simulink model "VirtualVehicle_Lab2_Soln"  (R2023b)
settings: Solver=VariableStepAuto  StartTime=0.0  StopTime=30  MaxStep=0.002  RelTol=1e-3
values from neighbouring files (symbols this model uses):
  m = 1000    [VehicleModelSoln.m]
  s = tf('s')    [PositionAnalysisSoln.m]
undefined symbols (not defined in the file or in its folder): X, Y, Z
libraries: sm_lib x59, nesl_utility x12, fl_lib x5, sdl_lib x1
(part 1 of 2)
settings Model: Creator=Rocksmithed  LastModifiedBy=callie
settings DebuggingCC: UnconnectedInputMsg=warning  UnconnectedOutputMsg=warning  UnconnectedLineMsg=warning
settings ModelReferenceCC: EnableRefExpFcnMdlSchedulingChecks=on
settings RTWCC: DLArmComputeVersion=19.05
settings SimscapeCC: SimscapeLogType=all  SimscapeLogLimitData=off
settings DiagnosticsConfigSet: SimMechanicsConflictingReferenceFrames=none
settings ExplorerConfigSet: InternalSimMechanicsExplorerSettings="<ExplorerConfiguration><canonicalview>default</canonicalview><AnimationSetting><BasePlaybackSpeed>1.0</BasePlaybackSpeed><PlaybackSpeedFactor>1.0</PlaybackSpeedFactor></AnimationSetting><TilePanel><TileInfo><Tiles Columns=\"1\" Count=\"2\" Rows=\"2\"><Column Weight=\"1\"/><Row Weight=\"0.4997\"/><Row Weight=\"0.5003\"/><Tile Height=\"1\" Width=\"1\" X=\"0\" Y=\"0\"/><Tile Height=\"1\" Width=\"1\" X=\"0\" Y=\"1\"/></Tiles></TileInfo><SceneInfo><SceneViewer><BGColor><R>0.800000011920928955</R><G>0.800000011920928955</G><B>0.800000011920928955</B></BGColor><Camera><DoPerspective>on</DoPerspective><Position><X>5.90000000000000036</X><Y>-6</Y><Z>6.75</Z></Position><Center><X>5.32642356364895431</X><Y>-5.37249312840286741</Y><Z>6.22345921548163616</Z></Center><Up><X>0</X><Y>0</Y><Z>1</Z></Up><ViewLimDist>1</ViewLimDist><YLim>0.466307658154998583</YLim><XLim>1.21820086771592928</XLim></Camera></SceneViewer><SceneViewer><BGColor><R>0.800000011920928955</R><G>0.800000011920928955</G><B>0.800000011920928955</B></BGColor><Camera><DoPerspective>on</DoPerspective><Position><X>-1</X><Y>-15</Y><Z>0</Z></Position><Center><X>-1</X><Y>-14</Y><Z>-2.22044604925031308e-16</Z></Center><Up><X>0</X><Y>0</Y><Z>1</Z></Up><ViewLimDist>1</ViewLimDist><YLim>0.466307658154998583</YLim><XLim>1.21239991120299639</XLim></Camera></SceneViewer></SceneInfo></TilePanel><MechEditorPanel><Cameras><Camera><Id>Camera1</Id><Value><Name>Camera Tracking Iso</Name><NativeCamera><PositionTrackingFeature>Vehicle_and_road.Animation.Cameras.Reference_Camera_Iso.R</PositionTrackingFeature><CenterTrackingFeature>Vehicle_and_road.Animation.Cameras.Reference_Camera_Iso.R</CenterTrackingFeature><UpVectorTrackingFeature>Vehicle_and_road.Animation.World_Frame.W</UpVectorTrackingFeature><CenterTrackingOrigin>off</CenterTrackingOrigin><CenterTrackingDirection>-Z</CenterTrackingDirection><UpVectorTrackingDirection>+Z</UpVectorTrackingDirection></NativeCamera></Value></Camera><Camera><Id>Camera2</Id><Value><Name>Camera Tracking Side</Name><NativeCamera><PositionTrackingFeature>Vehicle_and_road.Animation.Cameras.Reference_Camera_Side.R</PositionTrackingFeature><CenterTrackingFeature>Vehicle_and_road.Animation.Cameras.Reference_Camera_Side.R</CenterTrackingFeature><UpVectorTrackingFeature>Vehicle_and_road.Animation.World_Frame.W</UpVectorTrackingFeature><CenterTrackingOrigin>off</CenterTrackingOrigin><CenterTrackingDirection>-Z</CenterTrackingDirection><UpVectorTrackingDirection>+Z</UpVectorTrackingDirection></NativeCamera></Value></Camera></Cameras><GfxPanelCameraMap><MapElement CameraMLId=\"Camera1\" GfxPanelIndex=\"0\"/><MapElement CameraMLId=\"Camera2\" GfxPanelIndex=\"1\"/></GfxPanelCameraMap><VideoCreator><PlaybackSpeedRatio>1.0</PlaybackSpeedRatio><FrameRate>30</FrameRate><VideoFormat>Motion JPEG AVI</VideoFormat><FrameSize>auto</FrameSize></VideoCreator></MechEditorPanel></ExplorerConfiguration>"

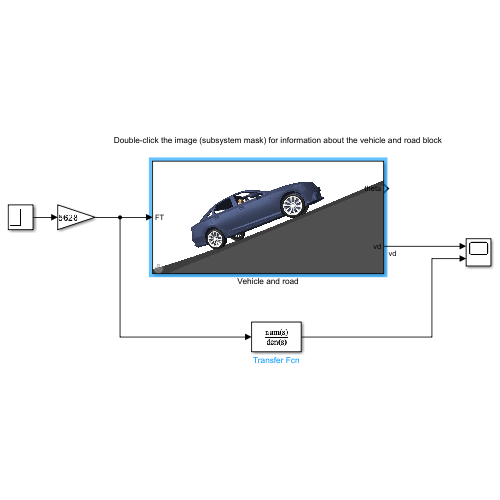
[thumbnail: Simulink's stored preview of the top-level diagram]
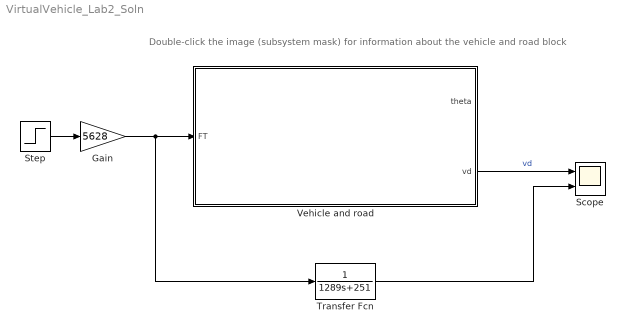
== system VirtualVehicle_Lab2_Soln ==
  note: Double-click the image (subsystem mask) for information about the vehicle and road block
  Gain : Gain  Gain=5628
  Scope : Scope  NumInputPorts=2
  Step : Step  Time=0  SampleTime=0
  Transfer Fcn : TransferFcn  Denominator=[1289 251]
  Vehicle and road : Subsystem  mask{MaxF=14800.0, brkok=on, dtype=none, randbumps=on, h=20.0, bumpspace=68.0}
      mask prompts: MaxF "Traction force saturation limit"; brkok "Allow braking"; dtype "Disturbance type"; randbumps "Randomize bumps"; h "Disturbance height (m)"; bumpspace "Bump spacing (m)"
      mask help:
      | This block provides a 2D implementation and visualization of a virtual vehicle.
      |
      | Inputs:
      |    FT: traction force in Newtons.
      | Outputs:
      |    theta: road grade at current position in radians.
      |    vd: velocity in the direction of travel in m/s (car frame).
      mask init:
      | L = 500; % Track length (meters)
      | tw = 10; % Transition width (meters)
      | ext = 600; % Extra at the end
      | depth = 0.25; % Road depth (meters)
      | N = 10e3;
      | 
      | roadw = 5; % road width (m)
      | 
      | markerFreq = 200; % marker every X points
      | markerw = 0.1; % marker width
      | markerd = 0.05; % marker depth
      | markerh = 1.5; % marker height
      | 
      | b_friction = 250; % Additional friction force coefficient (N*s/m)
      | 
      | if(dtype==2)
      |     xb = [-4,L/4,L/2-tw,...
      |       L/2+tw,L*3/4,L+ext];
      |     yf = @(x) (x > L/4).*(x < L/2).*((h/(L/4)).*(x-L/4)) ...
      |         + (x >= L/2).*(x < 3*L/4).*((-h/(L/4)).*(x-L/2) + h);
      |     yb = yf(xb);
      | 
      | elseif(dtype==3)
      |     bumpx = L/10:bumpspace/2:9*L/10;
      |     n = 1:numel(bumpx);
      |     xb = [-4,bumpx,L,L+ext];
      |     yb = [0,h/2*(1+(-1).^(n)),0,0];
      | 
      |     % Bump randomization
      |     if(randbumps)
      |         bh = rand(1,numel(bumpx)).*h/2.*(1+(-1).^(n));
      |         yb = [0,bh,0,0];
      |     end
      | 
      | else
      |     xb = [-4,L+ext];
      |     yb = xb*0;
      |     
      | end
      |     
      | % Vehicle position
      | xc = linspace(0,xb(end),N);
      | yc = pchip([0,xb(2:end)],[0,yb(2:end)],xc);
      | 
      | % Road position
      | x = linspace(xb(1),xb(end),N);
      | y = pchip(xb,yb,x);
      | x2 = [x(1),x,x(end)];
      | y2 = [-depth,y,-depth];
      | roadcs = [x2(end:-1:1);y2(end:-1:1)]';
      | 
      | % Markers
      | ix = 1:round(markerFreq):length(x);
      | xm1 = [x(ix)-markerd;x(ix)-markerd;x(ix)+markerd;x(ix)+markerd];
      | ym1 = [y(ix)*0;y(ix)+markerh;y(ix)+markerh;y(ix)*0];
      | xm = [xm1(1),xm1(:)',xm1(end)];
      | ym = [-depth,ym1(:)',-depth];
      | 
      | markercs = [xm(end:-1:1);ym(end:-1:1)]';
      | 
      | 
      | % Braking?
      | llim = 0;
      | if(brkok)
      |     llim = -inf;
      | end
      mask TypeOptions dtype: none | hill | bumps
      mask DialogControl Container3 Prompt: Vehicle
      mask DialogControl Container4 Prompt: Road
      mask Display: image('vehicle.png');
  wires:
  Step/1 -> Gain/1
  Vehicle and road/2(vd) -> Scope/1  "vd"
  Transfer Fcn/1 -> Scope/2
  Gain/1 -> Transfer Fcn/1, Vehicle and road/1(FT)

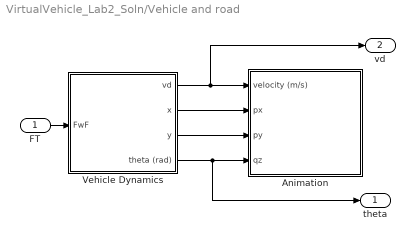
== system VirtualVehicle_Lab2_Soln/Vehicle and road ==
  FT : Inport
  Animation : Subsystem
  Vehicle Dynamics : Subsystem
  theta : Outport
  vd : Outport  Port=2
  wires:
  Vehicle Dynamics/1(vd) -> vd/1, Animation/1(velocity (m/s))
  FT/1 -> Vehicle Dynamics/1(FwF)
  Vehicle Dynamics/4(theta (rad)) -> theta/1, Animation/4(qz)
  Vehicle Dynamics/2(x) -> Animation/2(px)
  Vehicle Dynamics/3(y) -> Animation/3(py)

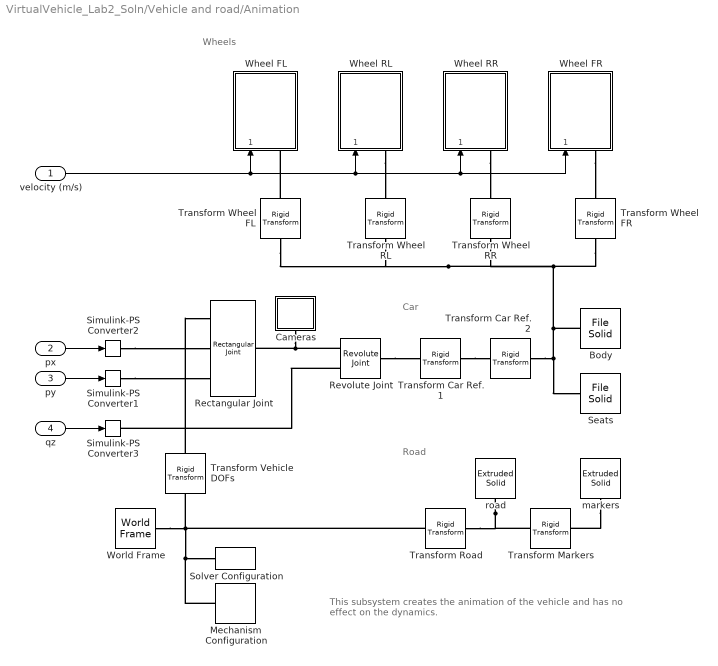
== system VirtualVehicle_Lab2_Soln/Vehicle and road/Animation ==
  note: This subsystem creates the animation of the vehicle and has no effect on the dynamics.
  note: Car
  note: Wheels
  note: Road
  velocity (m/s) : Inport
  px : Inport  Port=2
  py : Inport  Port=3
  qz : Inport  Port=4
  Body : sm_lib/Body Elements/File Solid  ExtGeomFileName=cc_Sedan_Hamba_body.STL  UnitType=Custom  ExtGeomFileUnits=mm  StepReaderType=HEX  ExportConvexHullGeometry=off  InertiaType=CalculateFromGeometry  Mass=1  MassUnits=kg  CenterOfMass=[0 0 0]  CenterOfMassUnits=m  MomentsOfInertia=[1 1 1]  MomentsOfInertiaUnits=kg*m^2  ProductsOfInertia=[0 0 0]  ProductsOfInertiaUnits=kg*m^2  BasedOnType=Density  Density=1000  DensityUnits=kg/m^3  DoExposeReferenceFrame=on  SerializedFrames=<Frames/>  GraphicType=FromGeometry  MarkerShape=Sphere  MarkerSize=10  GraphicVisPropType=AdvancedVisualProperties  GraphicDiffuseColor="[0.2670    0.3060    0.4270]"  GraphicSpecularColor="[0.2670    0.3060    0.4270]"  GraphicAmbientColor="[0.2670    0.3060    0.4270]/3"  GraphicEmissiveColor=[0 0 0]  GraphicShininess=20  GraphicOpacity=1.0
  Cameras : Subsystem
  Mechanism Configuration : sm_lib/Utilities/Mechanism Configuration  UniformGravity=Constant  GravityVector=[0 0 -9.80665*0]  GravityVectorUnits=m/s^2  GravityUnits=m/s^2  LinearizationDelta=0.001  JointModeTransitionNonlinearIterations=2
  Rectangular Joint : sm_lib/Joints/Rectangular Joint  JointMode=Normal  SenseConstraintForce=off  SenseConstraintForceX=off  SenseConstraintForceY=off  SenseConstraintForceZ=off  SenseConstraintTorque=off  SenseConstraintTorqueX=off  SenseConstraintTorqueY=off  SenseConstraintTorqueZ=off  SenseTotalForce=off  SenseTotalForceX=off  SenseTotalForceY=off  SenseTotalForceZ=off  SenseTotalTorque=off  SenseTotalTorqueX=off  SenseTotalTorqueY=off  SenseTotalTorqueZ=off  CompositeWrenchDir=FollowerOnBase  CompositeWrenchFrame=BaseFrame  PxEquilibriumPosition=0  PxEquilibriumPositionUnits=m  PxSpringStiffness=0  PxSpringStiffnessUnits=N/m  PxDampingCoefficient=0  PxDampingCoefficientUnits=N/(m/s)  PxTorqueActuationMode=ComputedTorque  PxMotionActuationMode=InputMotion  PxSensePosition=off  PxSenseVelocity=off  PxSenseAcceleration=off  PxSenseTorqueForce=off  PxSenseLowerLimitTorqueForce=off  PxSenseUpperLimitTorqueForce=off  PxLowerLimitSpecify=off  PxLowerLimitBound=-1  PxLowerLimitBoundUnits=m  PxLowerLimitStiffness=1e6  PxLowerLimitStiffnessUnits=N/m  PxLowerLimitDamping=1e3  PxLowerLimitDampingUnits=N/(m/s)  PxLowerLimitTransitionRegionWidth=1e-4  PxLowerLimitTransitionRegionWidthUnits=m  PxUpperLimitSpecify=off  PxUpperLimitBound=1  PxUpperLimitBoundUnits=m  PxUpperLimitStiffness=1e6  PxUpperLimitStiffnessUnits=N/m  PxUpperLimitDamping=1e3  PxUpperLimitDampingUnits=N/(m/s)  PxUpperLimitTransitionRegionWidth=1e-4  PxUpperLimitTransitionRegionWidthUnits=m  PxPositionTargetSpecify=off  PxPositionTargetPriority=High  PxPositionTargetValue=0  PxPositionTargetValueUnits=m  PxVelocityTargetSpecify=off  PxVelocityTargetPriority=High  PxVelocityTargetValue=0  PxVelocityTargetValueUnits=m/s  PyEquilibriumPosition=0  PyEquilibriumPositionUnits=m  PySpringStiffness=0  PySpringStiffnessUnits=N/m  PyDampingCoefficient=0  PyDampingCoefficientUnits=N/(m/s)  PyTorqueActuationMode=ComputedTorque  PyMotionActuationMode=InputMotion  PySensePosition=off  PySenseVelocity=off  PySenseAcceleration=off  PySenseTorqueForce=off  PySenseLowerLimitTorqueForce=off  PySenseUpperLimitTorqueForce=off  PyLowerLimitSpecify=off  PyLowerLimitBound=-1  PyLowerLimitBoundUnits=m  PyLowerLimitStiffness=1e6  PyLowerLimitStiffnessUnits=N/m  PyLowerLimitDamping=1e3  PyLowerLimitDampingUnits=N/(m/s)  PyLowerLimitTransitionRegionWidth=1e-4  PyLowerLimitTransitionRegionWidthUnits=m  PyUpperLimitSpecify=off  PyUpperLimitBound=1  PyUpperLimitBoundUnits=m  PyUpperLimitStiffness=1e6  PyUpperLimitStiffnessUnits=N/m  PyUpperLimitDamping=1e3  PyUpperLimitDampingUnits=N/(m/s)  PyUpperLimitTransitionRegionWidth=1e-4  PyUpperLimitTransitionRegionWidthUnits=m  PyPositionTargetSpecify=off  PyPositionTargetPriority=High  PyPositionTargetValue=0  PyPositionTargetValueUnits=m  PyVelocityTargetSpecify=off  PyVelocityTargetPriority=High  PyVelocityTargetValue=0  PyVelocityTargetValueUnits=m/s
  Revolute Joint : sm_lib/Joints/Revolute Joint  JointMode=Normal  SenseConstraintForce=off  SenseConstraintForceX=off  SenseConstraintForceY=off  SenseConstraintForceZ=off  SenseConstraintTorque=off  SenseConstraintTorqueX=off  SenseConstraintTorqueY=off  SenseConstraintTorqueZ=off  SenseTotalForce=off  SenseTotalForceX=off  SenseTotalForceY=off  SenseTotalForceZ=off  SenseTotalTorque=off  SenseTotalTorqueX=off  SenseTotalTorqueY=off  SenseTotalTorqueZ=off  CompositeWrenchDir=FollowerOnBase  CompositeWrenchFrame=BaseFrame  EquilibriumPosition=0  EquilibriumPositionUnits=deg  SpringStiffness=0  SpringStiffnessUnits=N*m/deg  DampingCoefficient=0  DampingCoefficientUnits=N*m/(deg/s)  TorqueActuationMode=ComputedTorque  MotionActuationMode=InputMotion  SensePosition=off  SenseVelocity=off  SenseAcceleration=off  SenseTorqueForce=off  SenseLowerLimitTorqueForce=off  SenseUpperLimitTorqueForce=off  LowerLimitSpecify=off  LowerLimitBound=-90  LowerLimitBoundUnits=deg  LowerLimitStiffness=1e4  LowerLimitStiffnessUnits=N*m/deg  LowerLimitDamping=10  LowerLimitDampingUnits=N*m/(deg/s)  LowerLimitTransitionRegionWidth=0.1  LowerLimitTransitionRegionWidthUnits=deg  UpperLimitSpecify=off  UpperLimitBound=90  UpperLimitBoundUnits=deg  UpperLimitStiffness=1e4  UpperLimitStiffnessUnits=N*m/deg  UpperLimitDamping=10  UpperLimitDampingUnits=N*m/(deg/s)  UpperLimitTransitionRegionWidth=0.1  UpperLimitTransitionRegionWidthUnits=deg  PositionTargetSpecify=off  PositionTargetPriority=High  PositionTargetValue=0  PositionTargetValueUnits=deg  VelocityTargetSpecify=off  VelocityTargetPriority=High  VelocityTargetValue=0  VelocityTargetValueUnits=deg/s
  Seats : sm_lib/Body Elements/File Solid  ExtGeomFileName=cc_Sedan_Hamba_seats.STL  UnitType=Custom  ExtGeomFileUnits=mm  StepReaderType=HEX  ExportConvexHullGeometry=off  InertiaType=CalculateFromGeometry  Mass=1  MassUnits=kg  CenterOfMass=[0 0 0]  CenterOfMassUnits=m  MomentsOfInertia=[1 1 1]  MomentsOfInertiaUnits=kg*m^2  ProductsOfInertia=[0 0 0]  ProductsOfInertiaUnits=kg*m^2  BasedOnType=Density  Density=1000  DensityUnits=kg/m^3  DoExposeReferenceFrame=on  SerializedFrames=<Frames/>  GraphicType=FromGeometry  MarkerShape=Sphere  MarkerSize=10  GraphicVisPropType=SimpleVisualProperties  GraphicDiffuseColor="[0.98 0.74  0.52]"  GraphicSpecularColor="[1    0.9   0.8 1]"  GraphicAmbientColor=[0.15 0.05 0.05 1]  GraphicEmissiveColor=[0.0 0.0 0.0 1.0]  GraphicShininess=25  GraphicOpacity=1.0
  Simulink-PS Converter1 : nesl_utility/Simulink-PS Converter  PhysicalDomain=network_engine_domain  SubClassName=ps_input  LeftPortType=input  RightPortType=output  PseudoPeriodic=off  Frequencies=[]  NoiseDistribution=none  NoiseParameters=[]  Unit=1  AffineConversion=off  FilteringAndDerivatives=filter  SimscapeFilterOrder=2  InputFilterTimeConstant=0.001  UdotUserProvided=0
  Simulink-PS Converter2 : nesl_utility/Simulink-PS Converter  PhysicalDomain=network_engine_domain  SubClassName=ps_input  LeftPortType=input  RightPortType=output  PseudoPeriodic=off  Frequencies=[]  NoiseDistribution=none  NoiseParameters=[]  Unit=1  AffineConversion=off  FilteringAndDerivatives=filter  SimscapeFilterOrder=2  InputFilterTimeConstant=0.001  UdotUserProvided=0
  Simulink-PS Converter3 : nesl_utility/Simulink-PS Converter  PhysicalDomain=network_engine_domain  SubClassName=ps_input  LeftPortType=input  RightPortType=output  PseudoPeriodic=off  Frequencies=[]  NoiseDistribution=none  NoiseParameters=[]  Unit=rad  AffineConversion=off  FilteringAndDerivatives=filter  SimscapeFilterOrder=2  InputFilterTimeConstant=0.001  UdotUserProvided=0
  Solver Configuration : nesl_utility/Solver Configuration  PhysicalDomain=network_engine_domain  SubClassName=solver  LeftPortType=input  RightPortType=generic  Tones=[]  Harmonics=[]  SimulateNoise=off  Profile=off  UseLocalSampling=off  EnableSwitchedLinearOptims=on  FrequencyDomain=off  UseCCode=off  RelTol=0.001  AbsTol=1e-06  MinStep=1e-09  ToWorkspace=off  RevertToSquareIcSolve=off  NumHomotopyIterations=100  PhasorMode=off  PhasorModeNumHarmonics=1  DoDC=off  ResidualTolerance=1e-09  UseLocalSolver=off  LocalSolverChoice=NE_BACKWARD_EULER_ADVANCER  LocalSolverSampleTime=0.001  DoFixedCost=off  MaxNonlinIter=3  MaxModeIter=2  ComputeImpulses=off  ImpulseIterations=2  LinearAlgebra=Sparse  EquationFormulation=NE_TIME_EF  DelaysMemoryBudget=1024  AutomaticFiltering=on  FilteringTimeConstant=0.001  PartitionStorageMethod=AS_NEEDED  PartitionMemoryBudget=1024  PartitionMethod=FAST
  Transform Car Ref. 1 : sm_lib/Frames and Transforms/Rigid Transform  TranslationMethod=None  TranslationStandardOffset=0  TranslationLengthUnit=m  TranslationStandardAxis=+Z  TranslationCartesianOffset=[0 0 0]  TranslationROffset=0  TranslationROffsetUnits=m  TranslationZOffset=0  TranslationZOffsetUnits=m  TranslationThetaOffset=0  TranslationThetaOffsetUnits=deg  RotationMethod=AlignedAxes  RotationAngleUnits=deg  RotationStandardAxis=+Z  RotationAngle=0.0  RotationArbitraryAxis=[0 0 1]  FollAlignAxisA=+Y  BaseAlignAxisA=+Z  FollAlignAxisB=+X  BaseAlignAxisB=+X  RotationSequenceAxes=FollowerAxes  RotationSequence=XYX  RotationSequenceAngles=[0 0 0]  RotationSequenceAnglesUnits=deg  RotationMatrix=[1 0 0; 0 1 0; 0 0 1]
  Transform Car Ref. 2 : sm_lib/Frames and Transforms/Rigid Transform  TranslationMethod=Cartesian  TranslationStandardOffset=0  TranslationLengthUnit=m  TranslationStandardAxis=+Z  TranslationCartesianOffset=[-4.1 -2 -3.25]  TranslationROffset=0  TranslationROffsetUnits=m  TranslationZOffset=0  TranslationZOffsetUnits=m  TranslationThetaOffset=0  TranslationThetaOffsetUnits=deg  RotationMethod=None  RotationAngleUnits=deg  RotationStandardAxis=+Z  RotationAngle=0.0  RotationArbitraryAxis=[0 0 1]  FollAlignAxisA=+X  BaseAlignAxisA=+Y  FollAlignAxisB=+Y  BaseAlignAxisB=+Z  RotationSequenceAxes=FollowerAxes  RotationSequence=XYX  RotationSequenceAngles=[0 0 0]  RotationSequenceAnglesUnits=deg  RotationMatrix=[1 0 0; 0 1 0; 0 0 1]
  Transform Markers : sm_lib/Frames and Transforms/Rigid Transform  TranslationMethod=StandardAxis  TranslationStandardOffset=-roadw/2-markerw  TranslationLengthUnit=m  TranslationStandardAxis=+Z  TranslationCartesianOffset=[0 0 0]  TranslationROffset=0  TranslationROffsetUnits=m  TranslationZOffset=0  TranslationZOffsetUnits=m  TranslationThetaOffset=0  TranslationThetaOffsetUnits=deg  RotationMethod=None  RotationAngleUnits=deg  RotationStandardAxis=+Z  RotationAngle=0.0  RotationArbitraryAxis=[0 0 1]  FollAlignAxisA=+X  BaseAlignAxisA=+Y  FollAlignAxisB=+Y  BaseAlignAxisB=+Z  RotationSequenceAxes=FollowerAxes  RotationSequence=XYX  RotationSequenceAngles=[0 0 0]  RotationSequenceAnglesUnits=deg  RotationMatrix=[1 0 0; 0 1 0; 0 0 1]
  Transform Road : sm_lib/Frames and Transforms/Rigid Transform  TranslationMethod=Cartesian  TranslationStandardOffset=0  TranslationLengthUnit=m  TranslationStandardAxis=+Z  TranslationCartesianOffset=[0 0 0]  TranslationROffset=0  TranslationROffsetUnits=m  TranslationZOffset=0  TranslationZOffsetUnits=m  TranslationThetaOffset=0  TranslationThetaOffsetUnits=deg  RotationMethod=AlignedAxes  RotationAngleUnits=deg  RotationStandardAxis=+Z  RotationAngle=0.0  RotationArbitraryAxis=[0 0 1]  FollAlignAxisA=+Z  BaseAlignAxisA=-Y  FollAlignAxisB=+Y  BaseAlignAxisB=+Z  RotationSequenceAxes=FollowerAxes  RotationSequence=XYX  RotationSequenceAngles=[0 0 0]  RotationSequenceAnglesUnits=deg  RotationMatrix=[1 0 0; 0 1 0; 0 0 1]
  Transform Vehicle DOFs : sm_lib/Frames and Transforms/Rigid Transform  TranslationMethod=Cartesian  TranslationStandardOffset=0  TranslationLengthUnit=m  TranslationStandardAxis=+Z  TranslationCartesianOffset=[0 0 0]  TranslationROffset=0  TranslationROffsetUnits=m  TranslationZOffset=0  TranslationZOffsetUnits=m  TranslationThetaOffset=0  TranslationThetaOffsetUnits=deg  RotationMethod=AlignedAxes  RotationAngleUnits=deg  RotationStandardAxis=+Z  RotationAngle=0.0  RotationArbitraryAxis=[0 0 1]  FollAlignAxisA=+Y  BaseAlignAxisA=+Z  FollAlignAxisB=+X  BaseAlignAxisB=+X  RotationSequenceAxes=FollowerAxes  RotationSequence=XYX  RotationSequenceAngles=[0 0 0]  RotationSequenceAnglesUnits=deg  RotationMatrix=[1 0 0; 0 1 0; 0 0 1]
  Transform Wheel FL : sm_lib/Frames and Transforms/Rigid Transform  TranslationMethod=None  TranslationStandardOffset=0  TranslationLengthUnit=m  TranslationStandardAxis=+Z  TranslationCartesianOffset=[0 0 0]  TranslationROffset=0  TranslationROffsetUnits=m  TranslationZOffset=0  TranslationZOffsetUnits=m  TranslationThetaOffset=0  TranslationThetaOffsetUnits=deg  RotationMethod=None  RotationAngleUnits=deg  RotationStandardAxis=+Z  RotationAngle=0.0  RotationArbitraryAxis=[0 0 1]  FollAlignAxisA=+X  BaseAlignAxisA=+Y  FollAlignAxisB=+Y  BaseAlignAxisB=+Z  RotationSequenceAxes=FollowerAxes  RotationSequence=XYX  RotationSequenceAngles=[0 0 0]  RotationSequenceAnglesUnits=deg  RotationMatrix=[1 0 0; 0 1 0; 0 0 1]
  Transform Wheel FR : sm_lib/Frames and Transforms/Rigid Transform  TranslationMethod=Cartesian  TranslationStandardOffset=0  TranslationLengthUnit=m  TranslationStandardAxis=+X  TranslationCartesianOffset=[8.22 4.4 0]  TranslationROffset=0  TranslationROffsetUnits=m  TranslationZOffset=0  TranslationZOffsetUnits=m  TranslationThetaOffset=0  TranslationThetaOffsetUnits=deg  RotationMethod=AlignedAxes  RotationAngleUnits=deg  RotationStandardAxis=+Z  RotationAngle=0.0  RotationArbitraryAxis=[0 0 1]  FollAlignAxisA=+Y  BaseAlignAxisA=-Y  FollAlignAxisB=+Z  BaseAlignAxisB=+Z  RotationSequenceAxes=FollowerAxes  RotationSequence=XYX  RotationSequenceAngles=[0 0 0]  RotationSequenceAnglesUnits=deg  RotationMatrix=[1 0 0; 0 1 0; 0 0 1]
  Transform Wheel RL : sm_lib/Frames and Transforms/Rigid Transform  TranslationMethod=Cartesian  TranslationStandardOffset=0  TranslationLengthUnit=m  TranslationStandardAxis=+Z  TranslationCartesianOffset=[-2.82 0 0]  TranslationROffset=0  TranslationROffsetUnits=m  TranslationZOffset=0  TranslationZOffsetUnits=m  TranslationThetaOffset=0  TranslationThetaOffsetUnits=deg  RotationMethod=None  RotationAngleUnits=deg  RotationStandardAxis=+Z  RotationAngle=0.0  RotationArbitraryAxis=[0 0 1]  FollAlignAxisA=+X  BaseAlignAxisA=+Y  FollAlignAxisB=+Y  BaseAlignAxisB=+Z  RotationSequenceAxes=FollowerAxes  RotationSequence=XYX  RotationSequenceAngles=[0 0 0]  RotationSequenceAnglesUnits=deg  RotationMatrix=[1 0 0; 0 1 0; 0 0 1]
  Transform Wheel RR : sm_lib/Frames and Transforms/Rigid Transform  TranslationMethod=Cartesian  TranslationStandardOffset=0  TranslationLengthUnit=m  TranslationStandardAxis=+X  TranslationCartesianOffset=[5.4 4.4 0]  TranslationROffset=0  TranslationROffsetUnits=m  TranslationZOffset=0  TranslationZOffsetUnits=m  TranslationThetaOffset=0  TranslationThetaOffsetUnits=deg  RotationMethod=AlignedAxes  RotationAngleUnits=deg  RotationStandardAxis=+Z  RotationAngle=0.0  RotationArbitraryAxis=[0 0 1]  FollAlignAxisA=+Y  BaseAlignAxisA=-Y  FollAlignAxisB=+Z  BaseAlignAxisB=+Z  RotationSequenceAxes=FollowerAxes  RotationSequence=XYX  RotationSequenceAngles=[0 0 0]  RotationSequenceAnglesUnits=deg  RotationMatrix=[1 0 0; 0 1 0; 0 0 1]
  Wheel FL : Subsystem
  Wheel FR : Subsystem
  Wheel RL : Subsystem
  Wheel RR : Subsystem
  World Frame : sm_lib/Frames and Transforms/World Frame
  markers : sm_lib/Body Elements/Extruded Solid  GraphicAmbientColor=[0.15 0.15 0.15 1.0]  BasedOnType=Density  CenterOfMass=[0 0 0]  CenterOfMassUnits=m  GraphicDiffuseColor=[1 0.9 0]  ExportConvexHullGeometry=off  ExtrusionCrossSection=markercs  ExtrusionCrossSectionUnits=m  Density=1000  DensityUnits=kg/m^3  DoExposeReferenceFrame=on  GraphicEmissiveColor=[0.0 0.0 0.0 1.0]  ExportEntireGeometry=off  ExtrusionLength=markerw  ExtrusionLengthUnits=m  ExtrusionType=General  SerializedFrames=<Frames/>  MarkerShape=Sphere  MarkerSize=10  GraphicType=FromGeometry  InertiaType=CalculateFromGeometry  Mass=1  MassUnits=kg  MomentsOfInertia=[1 1 1]  MomentsOfInertiaUnits=kg*m^2  PolygonNumSides=3  GraphicOpacity=1  PolygonOuterRadius=1  PolygonOuterRadiusUnits=m  ProductsOfInertia=[0 0 0]  ProductsOfInertiaUnits=kg*m^2  GraphicShininess=5  GraphicSpecularColor=[1 0.9 0]  GraphicVisPropType=SimpleVisualProperties
  road : sm_lib/Body Elements/Extruded Solid  GraphicAmbientColor=[0.15 0.15 0.15 1.0]  BasedOnType=Density  CenterOfMass=[0 0 0]  CenterOfMassUnits=m  GraphicDiffuseColor=[0.1 0.1 0.1]  ExportConvexHullGeometry=off  ExtrusionCrossSection=roadcs  ExtrusionCrossSectionUnits=m  Density=1000  DensityUnits=kg/m^3  DoExposeReferenceFrame=on  GraphicEmissiveColor=[0.0 0.0 0.0 1.0]  ExportEntireGeometry=off  ExtrusionLength=roadw  ExtrusionLengthUnits=m  ExtrusionType=General  SerializedFrames=<Frames/>  MarkerShape=Sphere  MarkerSize=10  GraphicType=FromGeometry  InertiaType=CalculateFromGeometry  Mass=1  MassUnits=kg  MomentsOfInertia=[1 1 1]  MomentsOfInertiaUnits=kg*m^2  PolygonNumSides=3  GraphicOpacity=1.0  PolygonOuterRadius=1  PolygonOuterRadiusUnits=m  ProductsOfInertia=[0 0 0]  ProductsOfInertiaUnits=kg*m^2  GraphicShininess=5  GraphicSpecularColor=[0.5 0.5 0.5 1.0]  GraphicVisPropType=AdvancedVisualProperties
  wires:
  velocity (m/s)/1 -> Wheel RL/1(velocity (m/s)), Wheel FR/1(velocity (m/s)), Wheel RR/1(velocity (m/s)), Wheel FL/1(velocity (m/s))
  px/1 -> Simulink-PS Converter2/1
  py/1 -> Simulink-PS Converter1/1
  qz/1 -> Simulink-PS Converter3/1
  connections:
  Wheel RL/LConn1 -- Transform Wheel RL/RConn1
  markers/RConn1 -- Transform Markers/RConn1
  Revolute Joint/LConn2 -- Simulink-PS Converter3/RConn1
  Wheel FR/LConn1 -- Transform Wheel FR/RConn1
  Wheel RR/LConn1 -- Transform Wheel RR/RConn1
  Revolute Joint/LConn1 -- Rectangular Joint/RConn1 -- Cameras/LConn1
  Transform Wheel FL/RConn1 -- Wheel FL/LConn1
  Transform Car Ref. 2/RConn1 -- Body/RConn1 -- Transform Wheel FR/LConn1 -- Transform Wheel FL/LConn1 -- Transform Wheel RL/LConn1 -- Transform Wheel RR/LConn1 -- Seats/RConn1
  World Frame/RConn1 -- Transform Road/LConn1 -- Mechanism Configuration/RConn1 -- Solver Configuration/RConn1 -- Transform Vehicle DOFs/LConn1
  road/RConn1 -- Transform Road/RConn1 -- Transform Markers/LConn1
  Transform Vehicle DOFs/RConn1 -- Rectangular Joint/LConn1
  Simulink-PS Converter2/RConn1 -- Rectangular Joint/LConn2
  Simulink-PS Converter1/RConn1 -- Rectangular Joint/LConn3
  Revolute Joint/RConn1 -- Transform Car Ref. 1/RConn1
  Transform Car Ref. 1/LConn1 -- Transform Car Ref. 2/LConn1

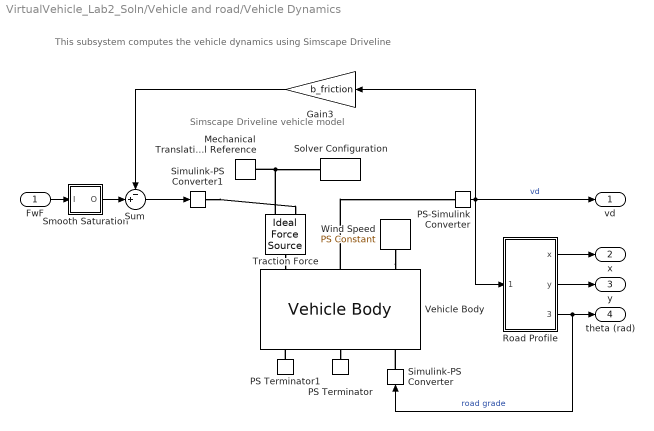
== system VirtualVehicle_Lab2_Soln/Vehicle and road/Vehicle Dynamics ==
  note: Simscape Driveline vehicle model
  note: This subsystem computes the vehicle dynamics using Simscape Driveline
  FwF : Inport
  Gain3 : Gain  Gain=b_friction
  Mechanical Translational Reference : fl_lib/Mechanical/Translational Elements/Mechanical Translational Reference
  PS Terminator : fl_lib/Physical Signals/Sinks/PS Terminator
  PS Terminator1 : fl_lib/Physical Signals/Sinks/PS Terminator
  PS-Simulink Converter : nesl_utility/PS-Simulink Converter  PhysicalDomain=network_engine_domain  SubClassName=ps_output  LeftPortType=input  RightPortType=output  PseudoPeriodic=off  Frequencies=[]  Unit=inherit  AffineConversion=off
  Road Profile : Subsystem
  Simulink-PS Converter : nesl_utility/Simulink-PS Converter  PhysicalDomain=network_engine_domain  SubClassName=ps_input  LeftPortType=input  RightPortType=output  PseudoPeriodic=off  Frequencies=[]  NoiseDistribution=none  NoiseParameters=[]  Unit=rad  AffineConversion=off  FilteringAndDerivatives=provide  SimscapeFilterOrder=1  InputFilterTimeConstant=0.001  UdotUserProvided=0
  Simulink-PS Converter1 : nesl_utility/Simulink-PS Converter  PhysicalDomain=network_engine_domain  SubClassName=ps_input  LeftPortType=input  RightPortType=output  PseudoPeriodic=off  Frequencies=[]  NoiseDistribution=none  NoiseParameters=[]  Unit=N  AffineConversion=off  FilteringAndDerivatives=provide  SimscapeFilterOrder=1  InputFilterTimeConstant=0.001  UdotUserProvided=0
  Smooth Saturation : Subsystem
  Solver Configuration : nesl_utility/Solver Configuration  PhysicalDomain=network_engine_domain  SubClassName=solver  LeftPortType=input  RightPortType=generic  Tones=[]  Harmonics=[]  SimulateNoise=off  Profile=off  UseLocalSampling=off  EnableSwitchedLinearOptims=on  FrequencyDomain=off  UseCCode=off  RelTol=0.001  AbsTol=1e-06  MinStep=1e-09  ToWorkspace=off  RevertToSquareIcSolve=off  NumHomotopyIterations=100  PhasorMode=off  PhasorModeNumHarmonics=1  DoDC=off  ResidualTolerance=1e-09  UseLocalSolver=off  LocalSolverChoice=NE_BACKWARD_EULER_ADVANCER  LocalSolverSampleTime=0.001  DoFixedCost=off  MaxNonlinIter=3  MaxModeIter=2  ComputeImpulses=off  ImpulseIterations=2  LinearAlgebra=auto  EquationFormulation=NE_TIME_EF  DelaysMemoryBudget=1024  AutomaticFiltering=on  FilteringTimeConstant=0.001  PartitionStorageMethod=AS_NEEDED  PartitionMemoryBudget=1024  PartitionMethod=ROBUST
  Sum : Sum  Inputs=-+|
  "Traction Force " : fl_lib/Mechanical/Mechanical Sources/Ideal Force Source
  Vehicle Body : sdl_lib/Tires & Vehicles/Vehicle Body  mass=1300 kg  n_w=2  x_f=1.4 m  x_r=1.8 m  y_c=.35 m  mass_var=simscape.enum.onoff.off  model_pitch=simscape.enum.onoff.off  inertia=4000 kg*m^2  suspension_model=sdl.enum.linearTLU.linear  k_f=1e4 N/m  b_f=1e4 N/(m/s)  k_r=1e4 N/m  b_r=1e4 N/(m/s)  k_f_TLU=[-2000, -1000, 0, 1000, 2000] N  x_f_TLU=[-.4, -.2, 0, .2, .4] m  b_f_TLU=[-200, -100, 0, 100, 200] N  v_f_TLU=[-4, -2, 0, 2, 4] m/s  k_r_TLU=[-2000, -1000, 0, 1000, 2000] N  x_r_TLU=[-.4, -.2, 0, .2, .4] m  b_r_TLU=[-200, -100, 0, 100, 200] N  v_r_TLU=[-4, -2, 0, 2, 4] m/s  interp_method=simscape.enum.interpolation.linear  extrap_method=simscape.enum.extrapolation.linear  model_hardstop=simscape.enum.onoff.off  upper_bound_f=.25 m  lower_bound_f=-.25 m  stop_k_f=1e6 N/m  stop_b_f=150 N/(m/s)  upper_bound_r=.25 m  lower_bound_r=-.25 m  stop_k_r=1e6 N/m  stop_b_r=150 N/(m/s)  initial_pitch=0 rad  initial_pitch_rate=0 rad/s  g=9.81 m/s^2  liftoff_warning=simscape.enum.onoff.off  area=6 m^2  Cd=0.6  rho=1.225 kg/m^3  v_specify=off  v_priority=High  v=0 m/s  v_nominal_specify=off  v_nominal_unit=m/s  v_nominal_value=1
  Wind Speed : fl_lib/Physical Signals/Sources/PS Constant  constant=0 m/s
  vd : Outport
  x : Outport  Port=2
  y : Outport  Port=3
  theta (rad) : Outport  Port=4
  wires:
  Gain3/1 -> Sum/1
  Sum/1 -> Simulink-PS Converter1/1
  PS-Simulink Converter/1 -> vd/1, Gain3/1, Road Profile/1(xdot)  "vd"
  Road Profile/3(theta (rad)) -> theta (rad)/1, Simulink-PS Converter/1  "road grade"
  Road Profile/1(x) -> x/1
  Road Profile/2(y) -> y/1
  FwF/1 -> Smooth Saturation/1(I)
  Smooth Saturation/1(O) -> Sum/2
  connections:
  "Traction Force "/LConn1 -- Vehicle Body/LConn1
  Vehicle Body/RConn2 -- PS Terminator/LConn1
  PS Terminator1/LConn1 -- Vehicle Body/RConn1
  "Traction Force "/RConn2 -- Mechanical Translational Reference/LConn1 -- Solver Configuration/RConn1
  Simulink-PS Converter/RConn1 -- Vehicle Body/RConn3
  Vehicle Body/LConn2 -- PS-Simulink Converter/LConn1
  Simulink-PS Converter1/RConn1 -- "Traction Force "/RConn1
  Wind Speed/RConn1 -- Vehicle Body/LConn3

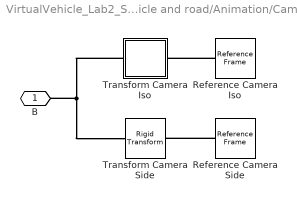
== system VirtualVehicle_Lab2_Soln/Vehicle and road/Animation/Cameras ==
  Reference Camera Iso : sm_lib/Frames and Transforms/Reference Frame
  Reference Camera Side : sm_lib/Frames and Transforms/Reference Frame
  Transform Camera Iso : Subsystem
  Transform Camera Side : sm_lib/Frames and Transforms/Rigid Transform  TranslationMethod=Cartesian  TranslationStandardOffset=0  TranslationLengthUnit=m  TranslationStandardAxis=+Z  TranslationCartesianOffset=[-1 0 15]  TranslationROffset=0  TranslationROffsetUnits=m  TranslationZOffset=0  TranslationZOffsetUnits=m  TranslationThetaOffset=0  TranslationThetaOffsetUnits=deg  RotationMethod=None  RotationAngleUnits=deg  RotationStandardAxis=+Z  RotationAngle=0.0  RotationArbitraryAxis=[0 0 1]  FollAlignAxisA=+X  BaseAlignAxisA=+Y  FollAlignAxisB=+Y  BaseAlignAxisB=+Z  RotationSequenceAxes=FollowerAxes  RotationSequence=XYZ  RotationSequenceAngles=[50 25 -80]  RotationSequenceAnglesUnits=deg  RotationMatrix=[1 0 0; 0 1 0; 0 0 1]
  B : PMIOPort  Side=Left
  connections:
  Reference Camera Side/RConn1 -- Transform Camera Side/RConn1
  Transform Camera Iso/LConn1 -- B/RConn1 -- Transform Camera Side/LConn1
  Reference Camera Iso/RConn1 -- Transform Camera Iso/RConn1

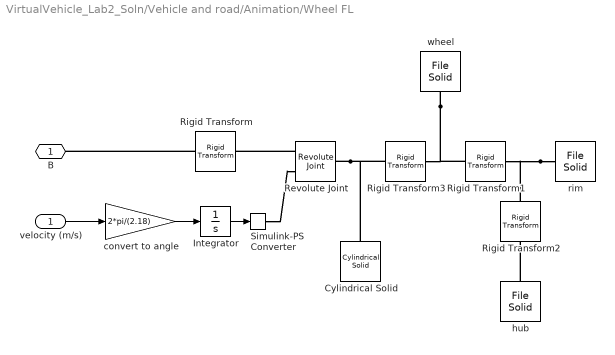
== system VirtualVehicle_Lab2_Soln/Vehicle and road/Animation/Wheel FL ==
  velocity (m/s) : Inport
  Cylindrical Solid : sm_lib/Body Elements/Cylindrical Solid  GraphicAmbientColor=[0.15 0.15 0.15 1.0]  BasedOnType=Mass  CenterOfMass=[0 0 0]  CenterOfMassUnits=m  GraphicDiffuseColor=[0.5 0.5 0.5]  CylinderLength=0.05  CylinderLengthUnits=m  CylinderRadius=0.05  CylinderRadiusUnits=m  Density=1000  DensityUnits=kg/m^3  DoExposeReferenceFrame=on  GraphicEmissiveColor=[0.0 0.0 0.0 1.0]  ExportEntireGeometry=off  SerializedFrames=<Frames/>  MarkerShape=Sphere  MarkerSize=10  GraphicType=FromGeometry  InertiaType=CalculateFromGeometry  Mass=10  MassUnits=kg  MomentsOfInertia=[1 1 1]  MomentsOfInertiaUnits=kg*m^2  GraphicOpacity=1.0  ProductsOfInertia=[0 0 0]  ProductsOfInertiaUnits=kg*m^2  GraphicShininess=75  GraphicSpecularColor=[0.5 0.5 0.5 1.0]  GraphicVisPropType=SimpleVisualProperties
  Integrator : Integrator
  Revolute Joint : sm_lib/Joints/Revolute Joint  JointMode=Normal  SenseConstraintForce=off  SenseConstraintForceX=off  SenseConstraintForceY=off  SenseConstraintForceZ=off  SenseConstraintTorque=off  SenseConstraintTorqueX=off  SenseConstraintTorqueY=off  SenseConstraintTorqueZ=off  SenseTotalForce=off  SenseTotalForceX=off  SenseTotalForceY=off  SenseTotalForceZ=off  SenseTotalTorque=off  SenseTotalTorqueX=off  SenseTotalTorqueY=off  SenseTotalTorqueZ=off  CompositeWrenchDir=FollowerOnBase  CompositeWrenchFrame=BaseFrame  EquilibriumPosition=0  EquilibriumPositionUnits=deg  SpringStiffness=0  SpringStiffnessUnits=N*m/deg  DampingCoefficient=0  DampingCoefficientUnits=N*m/(deg/s)  TorqueActuationMode=ComputedTorque  MotionActuationMode=InputMotion  SensePosition=off  SenseVelocity=off  SenseAcceleration=off  SenseTorqueForce=off  SenseLowerLimitTorqueForce=off  SenseUpperLimitTorqueForce=off  LowerLimitSpecify=off  LowerLimitBound=-90  LowerLimitBoundUnits=deg  LowerLimitStiffness=1e4  LowerLimitStiffnessUnits=N*m/deg  LowerLimitDamping=10  LowerLimitDampingUnits=N*m/(deg/s)  LowerLimitTransitionRegionWidth=0.1  LowerLimitTransitionRegionWidthUnits=deg  UpperLimitSpecify=off  UpperLimitBound=90  UpperLimitBoundUnits=deg  UpperLimitStiffness=1e4  UpperLimitStiffnessUnits=N*m/deg  UpperLimitDamping=10  UpperLimitDampingUnits=N*m/(deg/s)  UpperLimitTransitionRegionWidth=0.1  UpperLimitTransitionRegionWidthUnits=deg  PositionTargetSpecify=off  PositionTargetPriority=High  PositionTargetValue=0  PositionTargetValueUnits=deg  VelocityTargetSpecify=off  VelocityTargetPriority=High  VelocityTargetValue=-500  VelocityTargetValueUnits=deg/s
  Rigid Transform : sm_lib/Frames and Transforms/Rigid Transform  TranslationMethod=Cartesian  TranslationStandardOffset=0  TranslationLengthUnit=m  TranslationStandardAxis=+Z  TranslationCartesianOffset=[-4.112 -3.592 3]  TranslationROffset=0  TranslationROffsetUnits=m  TranslationZOffset=0  TranslationZOffsetUnits=m  TranslationThetaOffset=0  TranslationThetaOffsetUnits=deg  RotationMethod=AlignedAxes  RotationAngleUnits=deg  RotationStandardAxis=+Z  RotationAngle=0.0  RotationArbitraryAxis=[0 0 1]  FollAlignAxisA=+Z  BaseAlignAxisA=+Y  FollAlignAxisB=+X  BaseAlignAxisB=+X  RotationSequenceAxes=FollowerAxes  RotationSequence=XYX  RotationSequenceAngles=[0 0 0]  RotationSequenceAnglesUnits=deg  RotationMatrix=[1 0 0; 0 1 0; 0 0 1]
  Rigid Transform1 : sm_lib/Frames and Transforms/Rigid Transform  TranslationMethod=Cartesian  TranslationStandardOffset=0  TranslationLengthUnit=m  TranslationStandardAxis=+Z  TranslationCartesianOffset=[2.474 1.14 3.29]  TranslationROffset=0  TranslationROffsetUnits=m  TranslationZOffset=0  TranslationZOffsetUnits=m  TranslationThetaOffset=0  TranslationThetaOffsetUnits=deg  RotationMethod=AlignedAxes  RotationAngleUnits=deg  RotationStandardAxis=+Z  RotationAngle=0.0  RotationArbitraryAxis=[0 0 1]  FollAlignAxisA=+Z  BaseAlignAxisA=+Y  FollAlignAxisB=+X  BaseAlignAxisB=+X  RotationSequenceAxes=FollowerAxes  RotationSequence=XYX  RotationSequenceAngles=[0 0 0]  RotationSequenceAnglesUnits=deg  RotationMatrix=[1 0 0; 0 1 0; 0 0 1]
  Rigid Transform2 : sm_lib/Frames and Transforms/Rigid Transform  TranslationMethod=Cartesian  TranslationStandardOffset=0  TranslationLengthUnit=m  TranslationStandardAxis=+Z  TranslationCartesianOffset=[0 -0.57 0 ]  TranslationROffset=0  TranslationROffsetUnits=m  TranslationZOffset=0  TranslationZOffsetUnits=m  TranslationThetaOffset=0  TranslationThetaOffsetUnits=deg  RotationMethod=None  RotationAngleUnits=deg  RotationStandardAxis=+Z  RotationAngle=0.0  RotationArbitraryAxis=[0 0 1]  FollAlignAxisA=+X  BaseAlignAxisA=+Y  FollAlignAxisB=+Y  BaseAlignAxisB=+Z  RotationSequenceAxes=FollowerAxes  RotationSequence=XYX  RotationSequenceAngles=[0 0 0]  RotationSequenceAnglesUnits=deg  RotationMatrix=[1 0 0; 0 1 0; 0 0 1]
  Rigid Transform3 : sm_lib/Frames and Transforms/Rigid Transform  TranslationMethod=Cartesian  TranslationStandardOffset=0  TranslationLengthUnit=m  TranslationStandardAxis=+Z  TranslationCartesianOffset=[-4.112 -3.592 3]  TranslationROffset=0  TranslationROffsetUnits=m  TranslationZOffset=0  TranslationZOffsetUnits=m  TranslationThetaOffset=0  TranslationThetaOffsetUnits=deg  RotationMethod=AlignedAxes  RotationAngleUnits=deg  RotationStandardAxis=+Z  RotationAngle=0.0  RotationArbitraryAxis=[0 0 1]  FollAlignAxisA=+Z  BaseAlignAxisA=+Y  FollAlignAxisB=+X  BaseAlignAxisB=+X  RotationSequenceAxes=FollowerAxes  RotationSequence=XYX  RotationSequenceAngles=[0 0 0]  RotationSequenceAnglesUnits=deg  RotationMatrix=[1 0 0; 0 1 0; 0 0 1]
  Simulink-PS Converter : nesl_utility/Simulink-PS Converter  PhysicalDomain=network_engine_domain  SubClassName=ps_input  LeftPortType=input  RightPortType=output  PseudoPeriodic=off  Frequencies=[]  NoiseDistribution=none  NoiseParameters=[]  Unit=1  AffineConversion=off  FilteringAndDerivatives=filter  SimscapeFilterOrder=2  InputFilterTimeConstant=0.001  UdotUserProvided=0
  convert to angle : Gain  Gain=2*pi/(2.18)
  hub : sm_lib/Body Elements/File Solid  ExtGeomFileName=cc_Sedan_Hamba_wheel_hubcap.STEP  UnitType=Custom  ExtGeomFileUnits=mm  StepReaderType=HEX  ExportConvexHullGeometry=off  InertiaType=CalculateFromGeometry  Mass=0  MassUnits=kg  CenterOfMass=[0 0 0]  CenterOfMassUnits=m  MomentsOfInertia=[1 1 1]  MomentsOfInertiaUnits=kg*m^2  ProductsOfInertia=[0 0 0]  ProductsOfInertiaUnits=kg*m^2  BasedOnType=Mass  Density=1000  DensityUnits=kg/m^3  DoExposeReferenceFrame=on  SerializedFrames=<Frames/>  GraphicType=FromGeometry  MarkerShape=Sphere  MarkerSize=10  GraphicVisPropType=AdvancedVisualProperties  GraphicDiffuseColor=[1,1,1]  GraphicSpecularColor=[0.7 0.7 0.7]  GraphicAmbientColor=[0.2 0.2 0.2,1]  GraphicEmissiveColor=[0,0,0,1]  GraphicShininess=5  GraphicOpacity=1.0
  rim : sm_lib/Body Elements/File Solid  ExtGeomFileName=cc_Sedan_Hamba_wheel_rim.STEP  UnitType=Custom  ExtGeomFileUnits=mm  StepReaderType=HEX  ExportConvexHullGeometry=off  InertiaType=CalculateFromGeometry  Mass=0  MassUnits=kg  CenterOfMass=[0 0 0]  CenterOfMassUnits=m  MomentsOfInertia=[1 1 1]  MomentsOfInertiaUnits=kg*m^2  ProductsOfInertia=[0 0 0]  ProductsOfInertiaUnits=kg*m^2  BasedOnType=Mass  Density=1000  DensityUnits=kg/m^3  DoExposeReferenceFrame=on  SerializedFrames=<Frames/>  GraphicType=FromGeometry  MarkerShape=Sphere  MarkerSize=10  GraphicVisPropType=SimpleVisualProperties  GraphicDiffuseColor=[0.4 0.4 0.4]  GraphicSpecularColor="[1    0.9   0.8 1]"  GraphicAmbientColor=[0.15 0.05 0.05 1]  GraphicEmissiveColor=[0.0 0.0 0.0 1.0]  GraphicShininess=25  GraphicOpacity=1.0
  wheel : sm_lib/Body Elements/File Solid  ExtGeomFileName=cc_Sedan_Hamba_wheel_tire.STL  UnitType=Custom  ExtGeomFileUnits=mm  StepReaderType=HEX  ExportConvexHullGeometry=off  InertiaType=CalculateFromGeometry  Mass=0  MassUnits=kg  CenterOfMass=[0 0 0]  CenterOfMassUnits=m  MomentsOfInertia=[1 1 1]  MomentsOfInertiaUnits=kg*m^2  ProductsOfInertia=[0 0 0]  ProductsOfInertiaUnits=kg*m^2  BasedOnType=Mass  Density=0  DensityUnits=kg/m^3  DoExposeReferenceFrame=on  SerializedFrames=<Frames/>  GraphicType=FromGeometry  MarkerShape=Sphere  MarkerSize=10  GraphicVisPropType=SimpleVisualProperties  GraphicDiffuseColor=[0.2 0.2 0.2]  GraphicSpecularColor="[1    0.9   0.8 1]"  GraphicAmbientColor=[0.15 0.05 0.05 1]  GraphicEmissiveColor=[0.0 0.0 0.0 1.0]  GraphicShininess=25  GraphicOpacity=1.0
  B : PMIOPort  Side=Left
  wires:
  Integrator/1 -> Simulink-PS Converter/1
  convert to angle/1 -> Integrator/1
  velocity (m/s)/1 -> convert to angle/1
  connections:
  Simulink-PS Converter/RConn1 -- Revolute Joint/LConn2
  wheel/RConn1 -- Rigid Transform1/LConn1 -- Rigid Transform3/RConn1
  Revolute Joint/RConn1 -- Rigid Transform3/LConn1 -- Cylindrical Solid/RConn1
  Rigid Transform/RConn1 -- B/RConn1
  Revolute Joint/LConn1 -- Rigid Transform/LConn1
  hub/RConn1 -- Rigid Transform2/RConn1
  rim/RConn1 -- Rigid Transform2/LConn1 -- Rigid Transform1/RConn1

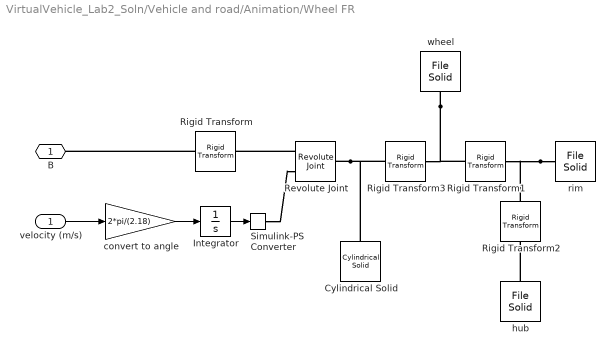
== system VirtualVehicle_Lab2_Soln/Vehicle and road/Animation/Wheel FR ==
  velocity (m/s) : Inport
  Cylindrical Solid : sm_lib/Body Elements/Cylindrical Solid  GraphicAmbientColor=[0.15 0.15 0.15 1.0]  BasedOnType=Mass  CenterOfMass=[0 0 0]  CenterOfMassUnits=m  GraphicDiffuseColor=[0.5 0.5 0.5]  CylinderLength=0.05  CylinderLengthUnits=m  CylinderRadius=0.05  CylinderRadiusUnits=m  Density=1000  DensityUnits=kg/m^3  DoExposeReferenceFrame=on  GraphicEmissiveColor=[0.0 0.0 0.0 1.0]  ExportEntireGeometry=off  SerializedFrames=<Frames/>  MarkerShape=Sphere  MarkerSize=10  GraphicType=FromGeometry  InertiaType=CalculateFromGeometry  Mass=10  MassUnits=kg  MomentsOfInertia=[1 1 1]  MomentsOfInertiaUnits=kg*m^2  GraphicOpacity=1.0  ProductsOfInertia=[0 0 0]  ProductsOfInertiaUnits=kg*m^2  GraphicShininess=75  GraphicSpecularColor=[0.5 0.5 0.5 1.0]  GraphicVisPropType=SimpleVisualProperties
  Integrator : Integrator
  Revolute Joint : sm_lib/Joints/Revolute Joint  JointMode=Normal  SenseConstraintForce=off  SenseConstraintForceX=off  SenseConstraintForceY=off  SenseConstraintForceZ=off  SenseConstraintTorque=off  SenseConstraintTorqueX=off  SenseConstraintTorqueY=off  SenseConstraintTorqueZ=off  SenseTotalForce=off  SenseTotalForceX=off  SenseTotalForceY=off  SenseTotalForceZ=off  SenseTotalTorque=off  SenseTotalTorqueX=off  SenseTotalTorqueY=off  SenseTotalTorqueZ=off  CompositeWrenchDir=FollowerOnBase  CompositeWrenchFrame=BaseFrame  EquilibriumPosition=0  EquilibriumPositionUnits=deg  SpringStiffness=0  SpringStiffnessUnits=N*m/deg  DampingCoefficient=0  DampingCoefficientUnits=N*m/(deg/s)  TorqueActuationMode=ComputedTorque  MotionActuationMode=InputMotion  SensePosition=off  SenseVelocity=off  SenseAcceleration=off  SenseTorqueForce=off  SenseLowerLimitTorqueForce=off  SenseUpperLimitTorqueForce=off  LowerLimitSpecify=off  LowerLimitBound=-90  LowerLimitBoundUnits=deg  LowerLimitStiffness=1e4  LowerLimitStiffnessUnits=N*m/deg  LowerLimitDamping=10  LowerLimitDampingUnits=N*m/(deg/s)  LowerLimitTransitionRegionWidth=0.1  LowerLimitTransitionRegionWidthUnits=deg  UpperLimitSpecify=off  UpperLimitBound=90  UpperLimitBoundUnits=deg  UpperLimitStiffness=1e4  UpperLimitStiffnessUnits=N*m/deg  UpperLimitDamping=10  UpperLimitDampingUnits=N*m/(deg/s)  UpperLimitTransitionRegionWidth=0.1  UpperLimitTransitionRegionWidthUnits=deg  PositionTargetSpecify=off  PositionTargetPriority=High  PositionTargetValue=0  PositionTargetValueUnits=deg  VelocityTargetSpecify=off  VelocityTargetPriority=High  VelocityTargetValue=-500  VelocityTargetValueUnits=deg/s
  Rigid Transform : sm_lib/Frames and Transforms/Rigid Transform  TranslationMethod=Cartesian  TranslationStandardOffset=0  TranslationLengthUnit=m  TranslationStandardAxis=+Z  TranslationCartesianOffset=[-4.112 -3.592 3]  TranslationROffset=0  TranslationROffsetUnits=m  TranslationZOffset=0  TranslationZOffsetUnits=m  TranslationThetaOffset=0  TranslationThetaOffsetUnits=deg  RotationMethod=AlignedAxes  RotationAngleUnits=deg  RotationStandardAxis=+Z  RotationAngle=0.0  RotationArbitraryAxis=[0 0 1]  FollAlignAxisA=+Z  BaseAlignAxisA=+Y  FollAlignAxisB=+X  BaseAlignAxisB=+X  RotationSequenceAxes=FollowerAxes  RotationSequence=XYX  RotationSequenceAngles=[0 0 0]  RotationSequenceAnglesUnits=deg  RotationMatrix=[1 0 0; 0 1 0; 0 0 1]
  Rigid Transform1 : sm_lib/Frames and Transforms/Rigid Transform  TranslationMethod=Cartesian  TranslationStandardOffset=0  TranslationLengthUnit=m  TranslationStandardAxis=+Z  TranslationCartesianOffset=[2.474 1.14 3.29]  TranslationROffset=0  TranslationROffsetUnits=m  TranslationZOffset=0  TranslationZOffsetUnits=m  TranslationThetaOffset=0  TranslationThetaOffsetUnits=deg  RotationMethod=AlignedAxes  RotationAngleUnits=deg  RotationStandardAxis=+Z  RotationAngle=0.0  RotationArbitraryAxis=[0 0 1]  FollAlignAxisA=+Z  BaseAlignAxisA=+Y  FollAlignAxisB=+X  BaseAlignAxisB=+X  RotationSequenceAxes=FollowerAxes  RotationSequence=XYX  RotationSequenceAngles=[0 0 0]  RotationSequenceAnglesUnits=deg  RotationMatrix=[1 0 0; 0 1 0; 0 0 1]
  Rigid Transform2 : sm_lib/Frames and Transforms/Rigid Transform  TranslationMethod=Cartesian  TranslationStandardOffset=0  TranslationLengthUnit=m  TranslationStandardAxis=+Z  TranslationCartesianOffset=[0 -0.57 0 ]  TranslationROffset=0  TranslationROffsetUnits=m  TranslationZOffset=0  TranslationZOffsetUnits=m  TranslationThetaOffset=0  TranslationThetaOffsetUnits=deg  RotationMethod=None  RotationAngleUnits=deg  RotationStandardAxis=+Z  RotationAngle=0.0  RotationArbitraryAxis=[0 0 1]  FollAlignAxisA=+X  BaseAlignAxisA=+Y  FollAlignAxisB=+Y  BaseAlignAxisB=+Z  RotationSequenceAxes=FollowerAxes  RotationSequence=XYX  RotationSequenceAngles=[0 0 0]  RotationSequenceAnglesUnits=deg  RotationMatrix=[1 0 0; 0 1 0; 0 0 1]
  Rigid Transform3 : sm_lib/Frames and Transforms/Rigid Transform  TranslationMethod=Cartesian  TranslationStandardOffset=0  TranslationLengthUnit=m  TranslationStandardAxis=+Z  TranslationCartesianOffset=[-4.112 -3.592 3]  TranslationROffset=0  TranslationROffsetUnits=m  TranslationZOffset=0  TranslationZOffsetUnits=m  TranslationThetaOffset=0  TranslationThetaOffsetUnits=deg  RotationMethod=AlignedAxes  RotationAngleUnits=deg  RotationStandardAxis=+Z  RotationAngle=0.0  RotationArbitraryAxis=[0 0 1]  FollAlignAxisA=+Z  BaseAlignAxisA=+Y  FollAlignAxisB=+X  BaseAlignAxisB=+X  RotationSequenceAxes=FollowerAxes  RotationSequence=XYX  RotationSequenceAngles=[0 0 0]  RotationSequenceAnglesUnits=deg  RotationMatrix=[1 0 0; 0 1 0; 0 0 1]
  Simulink-PS Converter : nesl_utility/Simulink-PS Converter  PhysicalDomain=network_engine_domain  SubClassName=ps_input  LeftPortType=input  RightPortType=output  PseudoPeriodic=off  Frequencies=[]  NoiseDistribution=none  NoiseParameters=[]  Unit=1  AffineConversion=off  FilteringAndDerivatives=filter  SimscapeFilterOrder=2  InputFilterTimeConstant=0.001  UdotUserProvided=0
  convert to angle : Gain  Gain=2*pi/(2.18)
  hub : sm_lib/Body Elements/File Solid  ExtGeomFileName=cc_Sedan_Hamba_wheel_hubcap.STEP  UnitType=Custom  ExtGeomFileUnits=mm  StepReaderType=HEX  ExportConvexHullGeometry=off  InertiaType=CalculateFromGeometry  Mass=0  MassUnits=kg  CenterOfMass=[0 0 0]  CenterOfMassUnits=m  MomentsOfInertia=[1 1 1]  MomentsOfInertiaUnits=kg*m^2  ProductsOfInertia=[0 0 0]  ProductsOfInertiaUnits=kg*m^2  BasedOnType=Mass  Density=1000  DensityUnits=kg/m^3  DoExposeReferenceFrame=on  SerializedFrames=<Frames/>  GraphicType=FromGeometry  MarkerShape=Sphere  MarkerSize=10  GraphicVisPropType=AdvancedVisualProperties  GraphicDiffuseColor=[1,1,1]  GraphicSpecularColor=[0.7 0.7 0.7]  GraphicAmbientColor=[0.2 0.2 0.2,1]  GraphicEmissiveColor=[0,0,0,1]  GraphicShininess=5  GraphicOpacity=1.0
  rim : sm_lib/Body Elements/File Solid  ExtGeomFileName=cc_Sedan_Hamba_wheel_rim.STEP  UnitType=Custom  ExtGeomFileUnits=mm  StepReaderType=HEX  ExportConvexHullGeometry=off  InertiaType=CalculateFromGeometry  Mass=0  MassUnits=kg  CenterOfMass=[0 0 0]  CenterOfMassUnits=m  MomentsOfInertia=[1 1 1]  MomentsOfInertiaUnits=kg*m^2  ProductsOfInertia=[0 0 0]  ProductsOfInertiaUnits=kg*m^2  BasedOnType=Mass  Density=1000  DensityUnits=kg/m^3  DoExposeReferenceFrame=on  SerializedFrames=<Frames/>  GraphicType=FromGeometry  MarkerShape=Sphere  MarkerSize=10  GraphicVisPropType=SimpleVisualProperties  GraphicDiffuseColor=[0.4 0.4 0.4]  GraphicSpecularColor="[1    0.9   0.8 1]"  GraphicAmbientColor=[0.15 0.05 0.05 1]  GraphicEmissiveColor=[0.0 0.0 0.0 1.0]  GraphicShininess=25  GraphicOpacity=1.0
  wheel : sm_lib/Body Elements/File Solid  ExtGeomFileName=cc_Sedan_Hamba_wheel_tire.STL  UnitType=Custom  ExtGeomFileUnits=mm  StepReaderType=HEX  ExportConvexHullGeometry=off  InertiaType=CalculateFromGeometry  Mass=0  MassUnits=kg  CenterOfMass=[0 0 0]  CenterOfMassUnits=m  MomentsOfInertia=[1 1 1]  MomentsOfInertiaUnits=kg*m^2  ProductsOfInertia=[0 0 0]  ProductsOfInertiaUnits=kg*m^2  BasedOnType=Mass  Density=0  DensityUnits=kg/m^3  DoExposeReferenceFrame=on  SerializedFrames=<Frames/>  GraphicType=FromGeometry  MarkerShape=Sphere  MarkerSize=10  GraphicVisPropType=SimpleVisualProperties  GraphicDiffuseColor=[0.2 0.2 0.2]  GraphicSpecularColor="[1    0.9   0.8 1]"  GraphicAmbientColor=[0.15 0.05 0.05 1]  GraphicEmissiveColor=[0.0 0.0 0.0 1.0]  GraphicShininess=25  GraphicOpacity=1.0
  B : PMIOPort  Side=Left
  wires:
  Integrator/1 -> Simulink-PS Converter/1
  convert to angle/1 -> Integrator/1
  velocity (m/s)/1 -> convert to angle/1
  connections:
  Simulink-PS Converter/RConn1 -- Revolute Joint/LConn2
  wheel/RConn1 -- Rigid Transform1/LConn1 -- Rigid Transform3/RConn1
  Revolute Joint/RConn1 -- Rigid Transform3/LConn1 -- Cylindrical Solid/RConn1
  Rigid Transform/RConn1 -- B/RConn1
  Revolute Joint/LConn1 -- Rigid Transform/LConn1
  hub/RConn1 -- Rigid Transform2/RConn1
  rim/RConn1 -- Rigid Transform2/LConn1 -- Rigid Transform1/RConn1
